simulink model "VF"  (R2023a)
settings: Solver=FixedStepAuto  StartTime=0.0  StopTime=10.0  FixedStep=0.00001  RelTol=1e-3
libraries: simulink x1
settings Model: Creator=35042  LastModifiedBy=35042

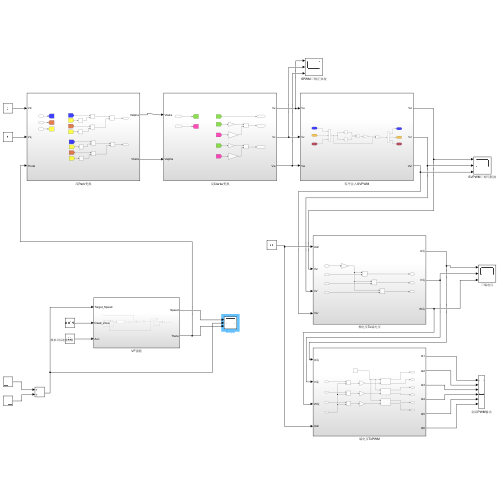
[thumbnail: Simulink's stored preview of the top-level diagram]
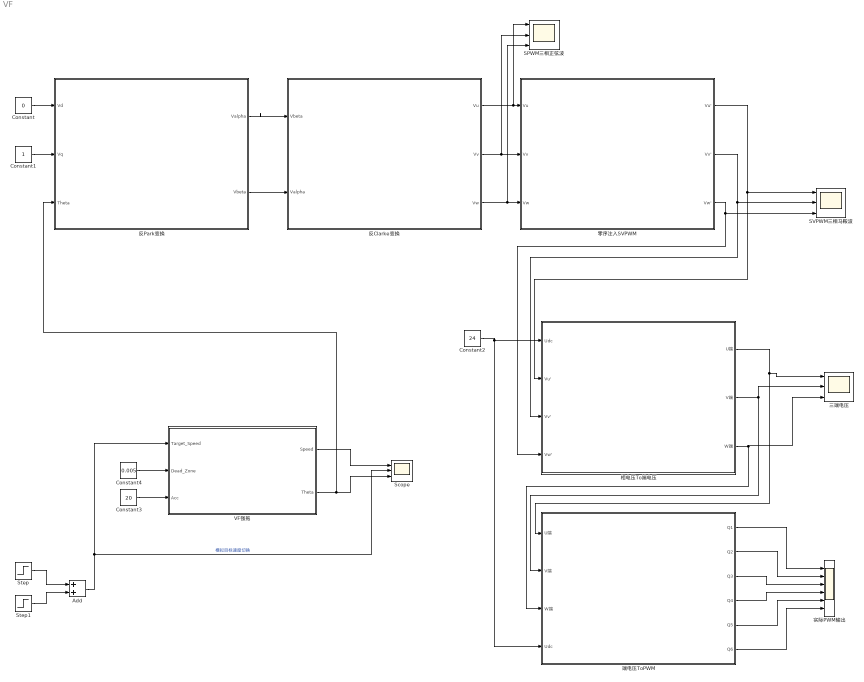
== system VF ==
  Add : Sum
  Constant : Constant  Value=0
  Constant1 : Constant
  Constant2 : Constant  Value=24
  Constant3 : Constant  Value=20
  Constant4 : Constant  Value=0.005
  SPWM三相正弦波 : Scope  NumInputPorts=3
  SVPWM三相马鞍波 : Scope  NumInputPorts=3
  Scope : Scope  NumInputPorts=3
  Step : Step  Time=0  After=50  SampleTime=0
  Step1 : Step  Time=5  After=-100  SampleTime=0
  VF强拖 : Subsystem
  三端电压 : Scope  NumInputPorts=3
  反Clarke变换 : Subsystem
  反Park变换 : Subsystem
  实际PWM输出 : Scope  NumInputPorts=6
  相电压To端电压 : Subsystem
  端电压ToPWM : Subsystem
  零序注入SVPWM : Subsystem
  wires:
  Constant/1 -> 反Park变换/1(Vd)
  Constant1/1 -> 反Park变换/2(Vq)
  反Park变换/1(Valpha) -> 反Clarke变换/1(Vbeta)
  反Park变换/2(Vbeta) -> 反Clarke变换/2(Valpha)
  反Clarke变换/1(Vu) -> SPWM三相正弦波/1, 零序注入SVPWM/1(Vu)
  反Clarke变换/2(Vv) -> SPWM三相正弦波/2, 零序注入SVPWM/2(Vv)
  反Clarke变换/3(Vw) -> 零序注入SVPWM/3(Vw), SPWM三相正弦波/3
  零序注入SVPWM/1(Vu') -> SVPWM三相马鞍波/1, 相电压To端电压/2(Vu')
  零序注入SVPWM/2(Vv') -> SVPWM三相马鞍波/2, 相电压To端电压/3(Vv')
  零序注入SVPWM/3(Vw') -> SVPWM三相马鞍波/3, 相电压To端电压/4(Vw')
  Constant2/1 -> 端电压ToPWM/4(Udc), 相电压To端电压/1(Udc)
  相电压To端电压/1(U端) -> 三端电压/1, 端电压ToPWM/1(U端)
  相电压To端电压/2(V端) -> 三端电压/2, 端电压ToPWM/2(V端)
  相电压To端电压/3(W端) -> 三端电压/3, 端电压ToPWM/3(W端)
  端电压ToPWM/1(Q1) -> 实际PWM输出/1
  端电压ToPWM/2(Q2) -> 实际PWM输出/2
  端电压ToPWM/3(Q3) -> 实际PWM输出/3
  端电压ToPWM/4(Q4) -> 实际PWM输出/4
  端电压ToPWM/5(Q5) -> 实际PWM输出/5
  端电压ToPWM/6(Q6) -> 实际PWM输出/6
  Constant4/1 -> VF强拖/2(Dead_Zone)
  Constant3/1 -> VF强拖/3(Acc)
  Step/1 -> Add/1
  Step1/1 -> Add/2
  Add/1 -> Scope/2, VF强拖/1(Target_Speed)  "模拟目标速度切换"
  VF强拖/1(Speed) -> Scope/1
  VF强拖/2(Theta) -> 反Park变换/3(Theta), Scope/3

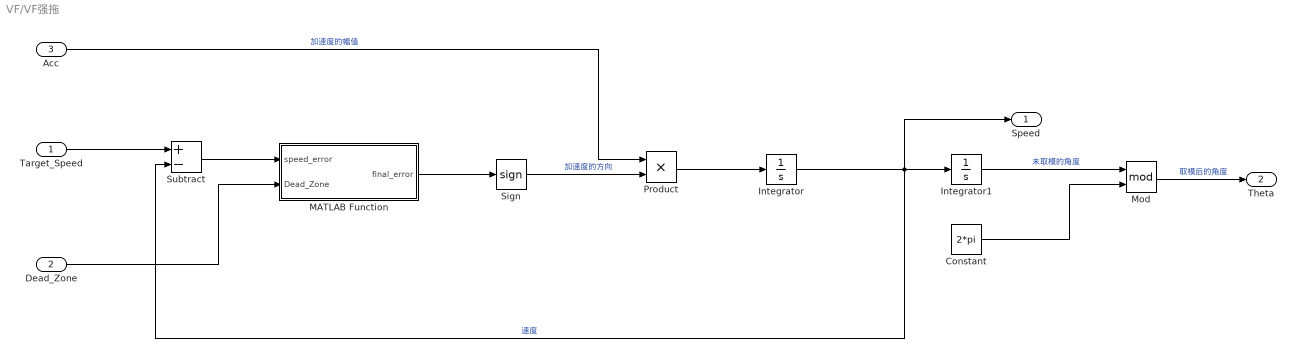
== system VF/VF强拖 ==
  Target_Speed : Inport
  Dead_Zone : Inport  Port=2
  Acc : Inport  Port=3
  Constant : Constant  Value=2*pi
  Integrator : Integrator
  Integrator1 : Integrator
  MATLAB Function : MATLAB Function  TreatAsAtomicUnit=on
  Mod : Math  Operator=mod
  Product : Product
  Sign : Signum
  Subtract : Sum  Inputs=+-
  Speed : Outport
  Theta : Outport  Port=2
  wires:
  Target_Speed/1 -> Subtract/1
  Subtract/1 -> MATLAB Function/1(speed_error)
  MATLAB Function/1(final_error) -> Sign/1
  Sign/1 -> Product/2  "加速度的方向"
  Acc/1 -> Product/1  "加速度的幅值"
  Dead_Zone/1 -> MATLAB Function/2(Dead_Zone)
  Product/1 -> Integrator/1
  Integrator/1 -> Speed/1, Subtract/2, Integrator1/1  "速度"
  Integrator1/1 -> Mod/1  "未取模的角度"
  Constant/1 -> Mod/2
  Mod/1 -> Theta/1  "取模后的角度"

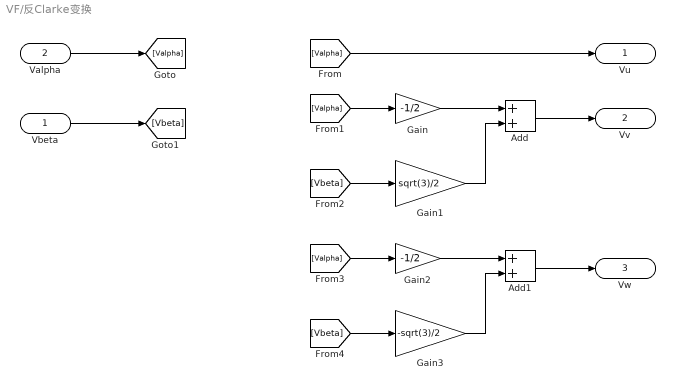
== system VF/反Clarke变换 ==
  Vbeta : Inport
  Valpha : Inport  Port=2
  Add : Sum
  Add1 : Sum
  Gain : Gain  Gain=-1/2
  Gain1 : Gain  Gain=sqrt(3)/2
  Gain2 : Gain  Gain=-1/2
  Gain3 : Gain  Gain=-sqrt(3)/2
  Vu : Outport
  Vv : Outport  Port=2
  Vw : Outport  Port=3
  wires:
  Valpha/1 -> [Valpha]
  Vbeta/1 -> [Vbeta]
  [Valpha] -> Vu/1
  [Valpha] -> Gain/1
  Gain/1 -> Add/1
  [Vbeta] -> Gain1/1
  Gain1/1 -> Add/2
  Add/1 -> Vv/1
  Gain2/1 -> Add1/1
  [Valpha] -> Gain2/1
  [Vbeta] -> Gain3/1
  Gain3/1 -> Add1/2
  Add1/1 -> Vw/1

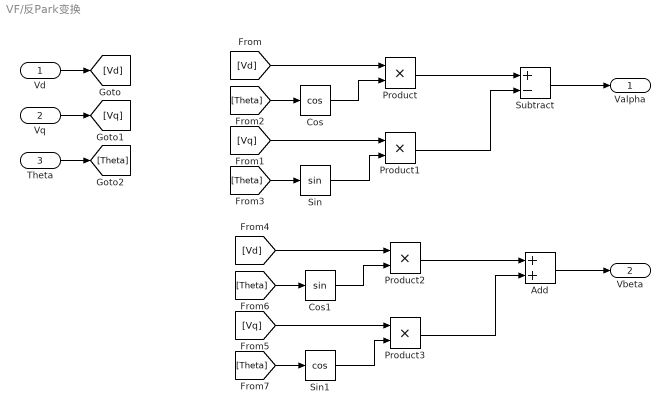
== system VF/反Park变换 ==
  Vd : Inport
  Vq : Inport  Port=2
  Theta : Inport  Port=3
  Add : Sum
  Cos : Trigonometry  Operator=cos
  Cos1 : Trigonometry
  Product{,1..3} (4 alike) : Product
  Sin : Trigonometry
  Sin1 : Trigonometry  Operator=cos
  Subtract : Sum  Inputs=+-
  Valpha : Outport
  Vbeta : Outport  Port=2
  wires:
  Vd/1 -> [Vd]
  Vq/1 -> [Vq]
  Theta/1 -> [Theta]
  [Theta] -> Cos/1
  [Vd] -> Product/1
  Cos/1 -> Product/2
  Product/1 -> Subtract/1
  [Vq] -> Product1/1
  [Theta] -> Sin/1
  Sin/1 -> Product1/2
  Product1/1 -> Subtract/2
  Subtract/1 -> Valpha/1
  [Vd] -> Product2/1
  Sin1/1 -> Product3/2
  Product2/1 -> Add/1
  Cos1/1 -> Product2/2
  [Theta] -> Sin1/1
  [Theta] -> Cos1/1
  [Vq] -> Product3/1
  Product3/1 -> Add/2
  Add/1 -> Vbeta/1

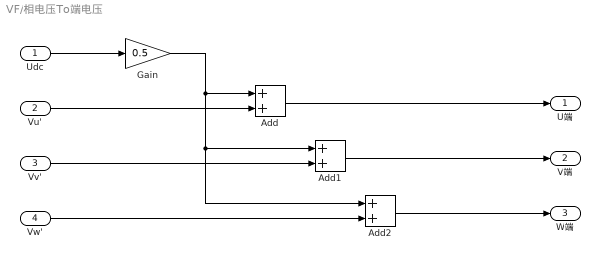
== system VF/相电压To端电压 ==
  Udc : Inport
  Vu' : Inport  Port=2
  Vv' : Inport  Port=3
  Vw' : Inport  Port=4
  Add : Sum
  Add1 : Sum
  Add2 : Sum
  Gain : Gain  Gain=0.5
  U端 : Outport
  V端 : Outport  Port=2
  W端 : Outport  Port=3
  wires:
  Udc/1 -> Gain/1
  Gain/1 -> Add2/1, Add1/1, Add/1
  Vu'/1 -> Add/2
  Add/1 -> U端/1
  Vv'/1 -> Add1/2
  Vw'/1 -> Add2/2
  Add2/1 -> W端/1
  Add1/1 -> V端/1

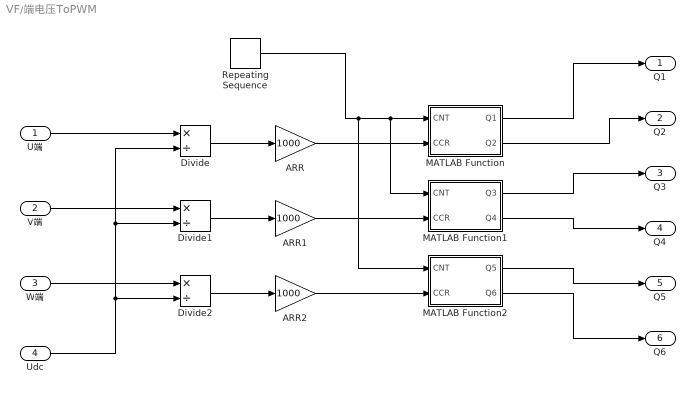
== system VF/端电压ToPWM ==
  U端 : Inport
  V端 : Inport  Port=2
  W端 : Inport  Port=3
  Udc : Inport  Port=4
  ARR : Gain  Gain=1000
  ARR1 : Gain  Gain=1000
  ARR2 : Gain  Gain=1000
  Divide : Product  Inputs=*/
  Divide1 : Product  Inputs=*/
  Divide2 : Product  Inputs=*/
  MATLAB Function : MATLAB Function  TreatAsAtomicUnit=on
  MATLAB Function1 : MATLAB Function  TreatAsAtomicUnit=on
  MATLAB Function2 : MATLAB Function  TreatAsAtomicUnit=on
  Repeating Sequence : simulink/Sources/Repeating Sequence  rep_seq_t=[0 0.0005 0.001]  rep_seq_y=[0 1000 0]
  Q1 : Outport
  Q2 : Outport  Port=2
  Q3 : Outport  Port=3
  Q4 : Outport  Port=4
  Q5 : Outport  Port=5
  Q6 : Outport  Port=6
  wires:
  U端/1 -> Divide/1
  Udc/1 -> Divide/2, Divide1/2, Divide2/2
  V端/1 -> Divide1/1
  W端/1 -> Divide2/1
  Divide2/1 -> ARR2/1
  Divide1/1 -> ARR1/1
  Divide/1 -> ARR/1
  ARR/1 -> MATLAB Function/2(CCR)
  ARR1/1 -> MATLAB Function1/2(CCR)
  ARR2/1 -> MATLAB Function2/2(CCR)
  Repeating Sequence/1 -> MATLAB Function2/1(CNT), MATLAB Function1/1(CNT), MATLAB Function/1(CNT)
  MATLAB Function/1(Q1) -> Q1/1
  MATLAB Function/2(Q2) -> Q2/1
  MATLAB Function1/1(Q3) -> Q3/1
  MATLAB Function1/2(Q4) -> Q4/1
  MATLAB Function2/1(Q5) -> Q5/1
  MATLAB Function2/2(Q6) -> Q6/1

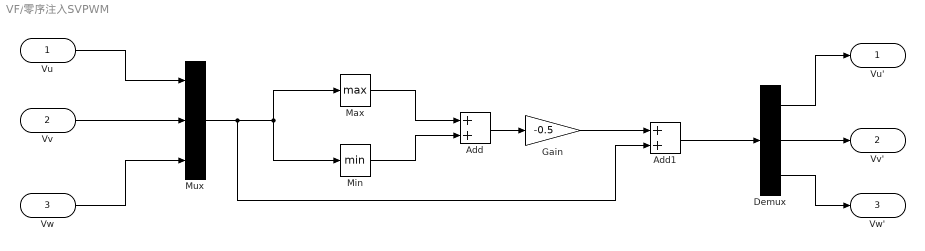
== system VF/零序注入SVPWM ==
  Vu : Inport
  Vv : Inport  Port=2
  Vw : Inport  Port=3
  Add : Sum
  Add1 : Sum
  Demux : Demux  Outputs=3
  Gain : Gain  Gain=-0.5
  Max : MinMax  Function=max
  Min : MinMax
  Mux : Mux  Inputs=3
  Vu' : Outport
  Vv' : Outport  Port=2
  Vw' : Outport  Port=3
  wires:
  Vu/1 -> Mux/1
  Vv/1 -> Mux/2
  Vw/1 -> Mux/3
  Mux/1 -> Add1/2, Min/1, Max/1
  Max/1 -> Add/1
  Min/1 -> Add/2
  Add/1 -> Gain/1
  Gain/1 -> Add1/1
  Add1/1 -> Demux/1
  Demux/1 -> Vu'/1
  Demux/2 -> Vv'/1
  Demux/3 -> Vw'/1

== matlab function VF/端电压ToPWM/MATLAB Function1 ==
  data: CNT input; CCR input; Q3 output; Q4 output
function [Q3,Q4] = fcn(CNT,CCR)

%初始化参数
Q3 = 0;
Q4 = 0;
if(CNT<=CCR)
    Q3 = 1;
    Q4 = 0;
elseif(CNT>CCR)
    Q3 = 0;
    Q4= 1;

end
end

== matlab function VF/端电压ToPWM/MATLAB Function ==
  data: CNT input; CCR input; Q1 output; Q2 output
function [Q1,Q2] = fcn(CNT,CCR)

%初始化参数
Q2 = 0;
Q1 = 0;
if(CNT<=CCR)
    Q1 = 1;
    Q2 = 0;
elseif(CNT>CCR)
    Q1 = 0;
    Q2= 1;

end
end

== matlab function VF/端电压ToPWM/MATLAB Function2 ==
  data: CNT input; CCR input; Q5 output; Q6 output
function [Q5,Q6] = fcn(CNT,CCR)

%初始化参数
Q5 = 0;
Q6 = 0;
if(CNT<=CCR)
    Q5 = 1;
    Q6 = 0;
elseif(CNT>CCR)
    Q5 = 0;
    Q6= 1;

end
end

== matlab function VF/VF强拖/MATLAB Function ==
  data: speed_error input; final_error output; Dead_Zone input
function final_error = fcn(speed_error, Dead_Zone)
if(abs(speed_error)<Dead_Zone)
    final_error = 0;
else 
    final_error = speed_error;
end

end
